simulink model "sf_lamp"  (R2025b)
settings: Solver=FixedStepDiscrete  StartTime=0.0  StopTime=10  FixedStep=0.01  RelTol=1e-3
libraries: simulink x1
settings Model: Creator=jbjtfy  LastModifiedBy=jbjtfy

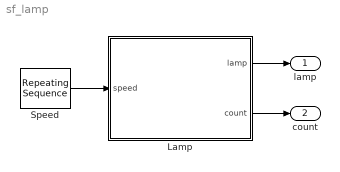
== system sf_lamp ==
  Lamp : Stateflow chart  TreatAsAtomicUnit=on
  Speed : simulink/Sources/Repeating Sequence  rep_seq_t=[0 4 8 10]  rep_seq_y=[0 80 0 0]
  lamp : Outport
  count : Outport  Port=2
  wires:
  Lamp/2(count) -> count/1
  Lamp/1(lamp) -> lamp/1
  Speed/1 -> Lamp/1(speed)

== stateflow chart sf_lamp/Lamp ==
  settings: updateMethod=DISCRETE  sampleTime=0.01
  state Off
    entry: lamp = 0;
  state On
    entry: lamp = 1;
  state Blinking
    entry: lamp = 2;
    during: count = count + 1;
  On -> Off [order 2] : [speed < 5]
  Blinking -> Off : [speed < 5]
  (default) -> Off : {lamp = 0; count = 0;}
  Off -> On : [speed > 10]
  On -> Blinking [order 1] : [speed > 50]
  data: speed input double; lamp output double =0; count output double =0
